simulink model "CasaDomotizadaModbus"  (R2024b)
settings: Solver=VariableStepAuto  StartTime=0.0  StopTime=100  RelTol=1e-3
undefined symbols (not defined in the file): localhost
libraries: modbuslib x4
settings Model: Creator=Ana  LastModifiedBy=Ana

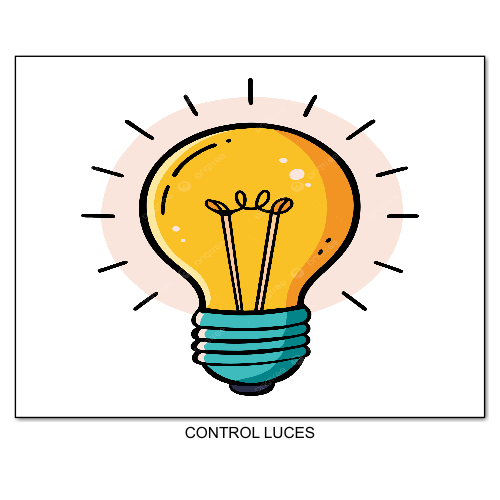
[thumbnail: Simulink's stored preview of the top-level diagram]
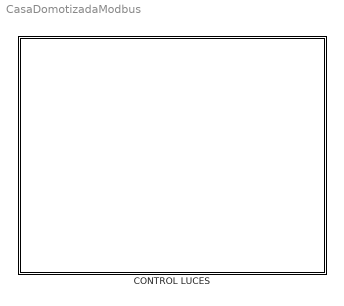
== system CasaDomotizadaModbus ==
  CONTROL LUCES : Subsystem
      mask Display: image('Bombilla.png');

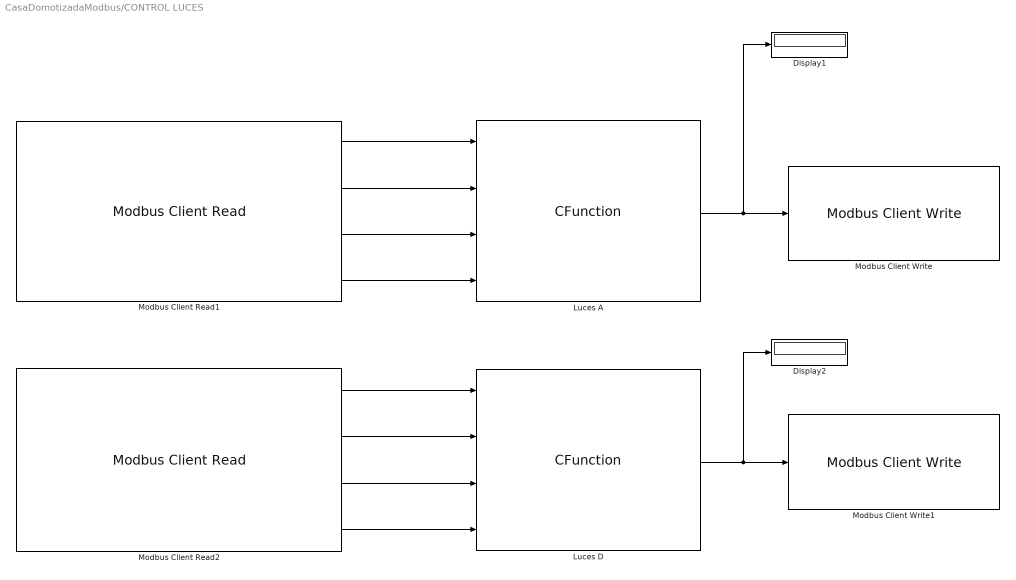
== system CasaDomotizadaModbus/CONTROL LUCES ==
  Display1 : Display
  Display2 : Display
  Luces A : CFunction  OutputCode=|  CodegenOutputCode=|  SampleTime=0.01
      OutputCode=|
      | int subir_actual = (A_DimmerSwitchUp > 0.5);
      | int bajar_actual = (A_DimmerSwitchDown > 0.5);
      | 
      | int flanco_subir = subir_actual && !subir_anterior;
      | 
      | int flanco_bajar = bajar_actual && !bajar_anterior;
      |     
      | subir_anterior = subir_actual;
      | bajar_anterior = bajar_actual;
      |     
      | /* Si el temporizador termina, 
      | apagar las luces*/
      | if (A_ActiveTimer < 0.5) {
      |     nivel_memorizado = 0.0;
      |     ciclo_iniciado = 0;
      | }
      | /* Si hay oscuridad y el temporizador está activo */
      | if (A_BrightnessCondition > 0.5 &&
      |     A_ActiveTimer > 0.5 && ciclo_iniciado == 0) {
      | 
      |     /* Primera activación: encender al nivel máximo */
      |         nivel_memorizado = 10.0;
      |         ciclo_iniciado = 1;
      |     }
      | if(ciclo_iniciado == 1){
      |         /* Ajustes manuales durante el temporizador */
      |         if (flanco_subir) {
      |             nivel_memorizado += 1.0;
      | 
      |             if (nivel_memorizado > 10.0) {
      |                 nivel_memorizado = 10.0;
      |             }
      |         }
      | 
      |         if (flanco_bajar) {
      |             nivel_memorizado -= 1.0;
      | 
      |             if (nivel_memorizado < 0.0) {
      |                 nivel_memorizado = 0.0;
      |             }
      |         }
      | }
      | 
      | 
      | /* Salida */
      | A_LightsAnalog = nivel_memorizado;
      CodegenOutputCode=|
      | int subir_actual = (A_DimmerSwitchUp > 0.5);
      | int bajar_actual = (A_DimmerSwitchDown > 0.5);
      | 
      | int flanco_subir = subir_actual && !subir_anterior;
      | 
      | int flanco_bajar = bajar_actual && !bajar_anterior;
      |     
      | subir_anterior = subir_actual;
      | bajar_anterior = bajar_actual;
      |     
      | /* Si el temporizador termina, 
      | apagar las luces*/
      | if (A_ActiveTimer < 0.5) {
      |     nivel_memorizado = 0.0;
      |     ciclo_iniciado = 0;
      | }
      | /* Si hay oscuridad y el temporizador está activo */
      | if (A_BrightnessCondition > 0.5 &&
      |     A_ActiveTimer > 0.5 && ciclo_iniciado == 0) {
      | 
      |     /* Primera activación: encender al nivel máximo */
      |         nivel_memorizado = 10.0;
      |         ciclo_iniciado = 1;
      |     }
      | if(ciclo_iniciado == 1){
      |         /* Ajustes manuales durante el temporizador */
      |         if (flanco_subir) {
      |             nivel_memorizado += 1.0;
      | 
      |             if (nivel_memorizado > 10.0) {
      |                 nivel_memorizado = 10.0;
      |             }
      |         }
      | 
      |         if (flanco_bajar) {
      |             nivel_memorizado -= 1.0;
      | 
      |             if (nivel_memorizado < 0.0) {
      |                 nivel_memorizado = 0.0;
      |             }
      |         }
      | }
      | 
      | 
      | /* Salida */
      | A_LightsAnalog = nivel_memorizado;
  Luces D : CFunction  OutputCode=|  CodegenOutputCode=|  SampleTime=0.01
      OutputCode=|
      | {
      | int subir_actual = (D_DimmerSwitchUp > 0.5);
      | int bajar_actual = (D_DimmerSwitchDown > 0.5);
      | 
      | int flanco_subir = subir_actual && !subir_anterior;
      | 
      | int flanco_bajar = bajar_actual && !bajar_anterior;
      |     
      | subir_anterior = subir_actual;
      | bajar_anterior = bajar_actual;
      |     
      | /* Si el temporizador termina, 
      | apagar las luces*/
      | if (D_ActiveTimer < 0.5) {
      |     nivel_memorizado = 0.0;
      |     ciclo_iniciado = 0;
      | }
      | /* Si hay oscuridad y el temporizador está activo */
      | if (D_BrightnessCondition > 0.5 &&
      |     D_ActiveTimer > 0.5 && ciclo_iniciado == 0) {
      | 
      |     /* Primera activación: encender al nivel máximo */
      |         nivel_memorizado = 10.0;
      |         ciclo_iniciado = 1;
      |     }
      | if(ciclo_iniciado == 1){
      |         /* Ajustes manuales durante el temporizador */
      |         if (flanco_subir) {
      |             nivel_memorizado += 1.0;
      | 
      |             if (nivel_memorizado > 10.0) {
      |                 nivel_memorizado = 10.0;
      |             }
      |         }
      | 
      |         if (flanco_bajar) {
      |             nivel_memorizado -= 1.0;
      | 
      |             if (nivel_memorizado < 0.0) {
      |                 nivel_memorizado = 0.0;
      |             }
      |         }
      | }
      | 
      | 
      | /* Salida */
      | D_LightsAnalog = nivel_memorizado;
      | }
      CodegenOutputCode=|
      | {
      | int subir_actual = (D_DimmerSwitchUp > 0.5);
      | int bajar_actual = (D_DimmerSwitchDown > 0.5);
      | 
      | int flanco_subir = subir_actual && !subir_anterior;
      | 
      | int flanco_bajar = bajar_actual && !bajar_anterior;
      |     
      | subir_anterior = subir_actual;
      | bajar_anterior = bajar_actual;
      |     
      | /* Si el temporizador termina, 
      | apagar las luces*/
      | if (D_ActiveTimer < 0.5) {
      |     nivel_memorizado = 0.0;
      |     ciclo_iniciado = 0;
      | }
      | /* Si hay oscuridad y el temporizador está activo */
      | if (D_BrightnessCondition > 0.5 &&
      |     D_ActiveTimer > 0.5 && ciclo_iniciado == 0) {
      | 
      |     /* Primera activación: encender al nivel máximo */
      |         nivel_memorizado = 10.0;
      |         ciclo_iniciado = 1;
      |     }
      | if(ciclo_iniciado == 1){
      |         /* Ajustes manuales durante el temporizador */
      |         if (flanco_subir) {
      |             nivel_memorizado += 1.0;
      | 
      |             if (nivel_memorizado > 10.0) {
      |                 nivel_memorizado = 10.0;
      |             }
      |         }
      | 
      |         if (flanco_bajar) {
      |             nivel_memorizado -= 1.0;
      | 
      |             if (nivel_memorizado < 0.0) {
      |                 nivel_memorizado = 0.0;
      |             }
      |         }
      | }
      | 
      | 
      | /* Salida */
      | D_LightsAnalog = nivel_memorizado;
      | }
  Modbus Client Read1 : modbuslib/Modbus Client Read  RetainClient=Salon_A_Client  ClientList=Salon_A_Client  ConnectionEndpoint=localhost:502  ServerId=1  RegisterTable={ '1', 'A_BrightnessCondition', '1', 'Input', 'bit', '1'; '2', 'A_ActiveTimer', '2', 'Input', 'bit', '1'; '3', 'A_DimmerSwitchUp', '3', 'Input', 'bit', '1'; '4', 'A_DimmerSwitchDown', '4', 'Input', 'bit', '1' }  SampleTime=0.01
  Modbus Client Read2 : modbuslib/Modbus Client Read  RetainClient=Salon_D_Client  ClientList=Salon_D_Client  ConnectionEndpoint=localhost:503  ServerId=1  RegisterTable={ '1', 'D_BrightnessCondition', '1', 'Input', 'bit', '1'; '2', 'D_ActiveTimer', '2', 'Input', 'bit', '1'; '3', 'D_DimmerSwitchUp', '3', 'Input', 'bit', '1'; '4', 'D_DimmerSwitchDown', '4', 'Input', 'bit', '1' }  SampleTime=0.01
  Modbus Client Write : modbuslib/Modbus Client Write  RetainClient=Salon_A_Client  ClientList=Salon_A_Client  ConnectionEndpoint=localhost:502  ServerId=1  RegisterTable={ '1', 'A_LightsAnalog', '1', 'Holding Register', 'uint16' }  SampleTime=0.01
  Modbus Client Write1 : modbuslib/Modbus Client Write  RetainClient=Salon_D_Client  ClientList=Salon_D_Client  ConnectionEndpoint=localhost:503  ServerId=1  RegisterTable={ '1', 'D_LightsAnalog', '1', 'Holding Register', 'uint16' }  SampleTime=0.01
  wires:
  Luces D/1 -> Modbus Client Write1/1, Display2/1
  Modbus Client Read2/1 -> Luces D/1
  Luces A/1 -> Display1/1, Modbus Client Write/1
  Modbus Client Read2/3 -> Luces D/3
  Modbus Client Read1/2 -> Luces A/2
  Modbus Client Read1/1 -> Luces A/1
  Modbus Client Read1/3 -> Luces A/3
  Modbus Client Read1/4 -> Luces A/4
  Modbus Client Read2/2 -> Luces D/2
  Modbus Client Read2/4 -> Luces D/4
